simulink model "DCHR_Earliest_Dispatch_Stateflow_v79"  (R2026a)
settings: Solver=FixedStepDiscrete  StopTime=0  FixedStep=1
model workspace (MAT data in the model file):
  dispatch_cfg_v66 = [0 0.2 20 70 48 60 0.01 0.9 0.8 40 4 30 35 5 5 0.5 0.5 2 5 45 2 0.1 0.25 0.25 2 68]
  dispatch_input_v66 = [0 1 0 0.1 0 0.1 0 0 0 0 3 0 1]
settings Model: Creator=Lysda  LastModifiedBy=Lysda

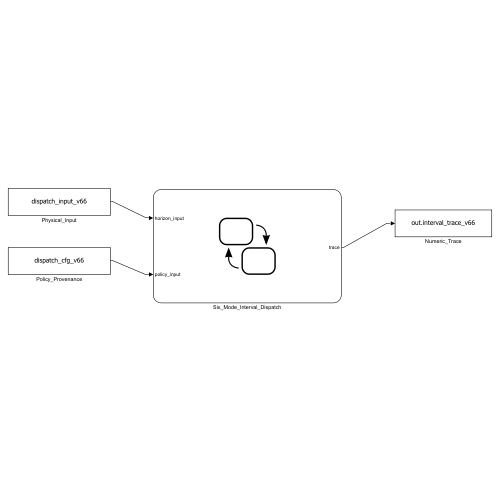
[thumbnail: Simulink's stored preview of the top-level diagram]
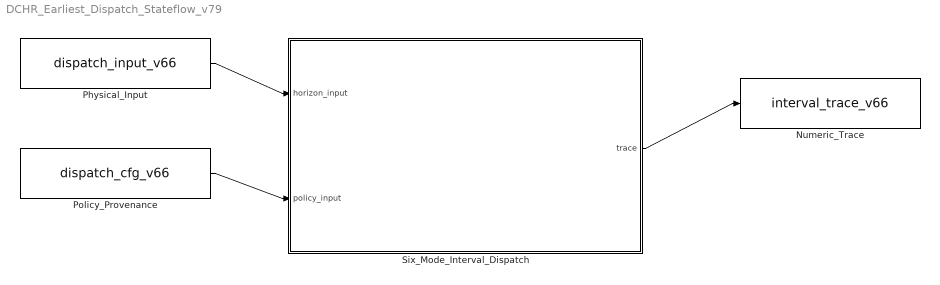
== system DCHR_Earliest_Dispatch_Stateflow_v79 ==
  Numeric_Trace : ToWorkspace  VariableName=interval_trace_v66  SaveFormat=Timeseries  SampleTime=-1
  Physical_Input : FromWorkspace  VariableName=dispatch_input_v66  SampleTime=1  Interpolate=off  OutputAfterFinalValue=Holding final value
  Policy_Provenance : FromWorkspace  VariableName=dispatch_cfg_v66  SampleTime=1  Interpolate=off  OutputAfterFinalValue=Holding final value
  Six_Mode_Interval_Dispatch : Stateflow chart  TreatAsAtomicUnit=on
  wires:
  Physical_Input/1 -> Six_Mode_Interval_Dispatch/1(horizon_input)
  Policy_Provenance/1 -> Six_Mode_Interval_Dispatch/2(policy_input)
  Six_Mode_Interval_Dispatch/1(trace) -> Numeric_Trace/1

== stateflow chart DCHR_Earliest_Dispatch_Stateflow_v79/Six_Mode_Interval_Dispatch ==
  settings: description=v79 pre-commit HP partition/energy/temporal-monitored SAME six-mode chart executes analytic earliest-event segments. Root hulls, symbolic thresholds, port offsets and physical clock survive each segment. No root midpoint. Macro solver ticks are protocol calls, not physical event times.
  state IDLE
    en:
    core=earliest_dispatch_kernel_v75(horizon_input,policy_input,retained_memory);
    assert(core(1)==0);
    monitor_hp_partition_v79(horizon_input,policy_input,retained_memory,core);
    trace=core;
    retained_memory=core;
    du:
    core=earliest_dispatch_kernel_v75(horizon_input,policy_input,retained_memory);
    assert(core(1)==0);
    monitor_hp_partition_v79(horizon_input,policy_input,retained_memory,core);
    trace=core;
    retained_memory=core;
  state HEAT_RECOVERY
    en:
    core=earliest_dispatch_kernel_v75(horizon_input,policy_input,retained_memory);
    assert(core(1)==1);
    monitor_hp_partition_v79(horizon_input,policy_input,retained_memory,core);
    trace=core;
    retained_memory=core;
    du:
    core=earliest_dispatch_kernel_v75(horizon_input,policy_input,retained_memory);
    assert(core(1)==1);
    monitor_hp_partition_v79(horizon_input,policy_input,retained_memory,core);
    trace=core;
    retained_memory=core;
  state STORAGE_CHARGE
    en:
    core=earliest_dispatch_kernel_v75(horizon_input,policy_input,retained_memory);
    assert(core(1)==2);
    monitor_hp_partition_v79(horizon_input,policy_input,retained_memory,core);
    trace=core;
    retained_memory=core;
    du:
    core=earliest_dispatch_kernel_v75(horizon_input,policy_input,retained_memory);
    assert(core(1)==2);
    monitor_hp_partition_v79(horizon_input,policy_input,retained_memory,core);
    trace=core;
    retained_memory=core;
  state STORAGE_DISCHARGE
    en:
    core=earliest_dispatch_kernel_v75(horizon_input,policy_input,retained_memory);
    assert(core(1)==3);
    monitor_hp_partition_v79(horizon_input,policy_input,retained_memory,core);
    trace=core;
    retained_memory=core;
    du:
    core=earliest_dispatch_kernel_v75(horizon_input,policy_input,retained_memory);
    assert(core(1)==3);
    monitor_hp_partition_v79(horizon_input,policy_input,retained_memory,core);
    trace=core;
    retained_memory=core;
  state BACKUP
    en:
    core=earliest_dispatch_kernel_v75(horizon_input,policy_input,retained_memory);
    assert(core(1)==4);
    monitor_hp_partition_v79(horizon_input,policy_input,retained_memory,core);
    trace=core;
    retained_memory=core;
    du:
    core=earliest_dispatch_kernel_v75(horizon_input,policy_input,retained_memory);
    assert(core(1)==4);
    monitor_hp_partition_v79(horizon_input,policy_input,retained_memory,core);
    trace=core;
    retained_memory=core;
  state UNMET_DEMAND
    en:
    core=earliest_dispatch_kernel_v75(horizon_input,policy_input,retained_memory);
    assert(core(1)==5);
    monitor_hp_partition_v79(horizon_input,policy_input,retained_memory,core);
    trace=core;
    retained_memory=core;
    du:
    core=earliest_dispatch_kernel_v75(horizon_input,policy_input,retained_memory);
    assert(core(1)==5);
    monitor_hp_partition_v79(horizon_input,policy_input,retained_memory,core);
    trace=core;
    retained_memory=core;
  (junction 60) -> UNMET_DEMAND [order 6] : [earliest_mode_v73(horizon_input,policy_input,retained_memory)==5]
  (junction 60) -> BACKUP [order 5] : [earliest_mode_v73(horizon_input,policy_input,retained_memory)==4]
  (junction 60) -> STORAGE_DISCHARGE [order 4] : [earliest_mode_v73(horizon_input,policy_input,retained_memory)==3]
  (junction 60) -> STORAGE_CHARGE [order 3] : [earliest_mode_v73(horizon_input,policy_input,retained_memory)==2]
  (junction 60) -> HEAT_RECOVERY [order 2] : [earliest_mode_v73(horizon_input,policy_input,retained_memory)==1]
  (default) -> (junction 60)
  (junction 60) -> IDLE [order 1] : [earliest_mode_v73(horizon_input,policy_input,retained_memory)==0]
  UNMET_DEMAND -> IDLE [order 1] : [earliest_mode_v73(horizon_input,policy_input,retained_memory)==0]
  BACKUP -> IDLE [order 1] : [earliest_mode_v73(horizon_input,policy_input,retained_memory)==0]
  STORAGE_DISCHARGE -> IDLE [order 1] : [earliest_mode_v73(horizon_input,policy_input,retained_memory)==0]
  STORAGE_CHARGE -> IDLE [order 1] : [earliest_mode_v73(horizon_input,policy_input,retained_memory)==0]
  HEAT_RECOVERY -> IDLE [order 1] : [earliest_mode_v73(horizon_input,policy_input,retained_memory)==0]
  UNMET_DEMAND -> HEAT_RECOVERY [order 2] : [earliest_mode_v73(horizon_input,policy_input,retained_memory)==1]
  BACKUP -> HEAT_RECOVERY [order 2] : [earliest_mode_v73(horizon_input,policy_input,retained_memory)==1]
  STORAGE_DISCHARGE -> HEAT_RECOVERY [order 2] : [earliest_mode_v73(horizon_input,policy_input,retained_memory)==1]
  STORAGE_CHARGE -> HEAT_RECOVERY [order 2] : [earliest_mode_v73(horizon_input,policy_input,retained_memory)==1]
  IDLE -> HEAT_RECOVERY [order 1] : [earliest_mode_v73(horizon_input,policy_input,retained_memory)==1]
  IDLE -> STORAGE_CHARGE [order 2] : [earliest_mode_v73(horizon_input,policy_input,retained_memory)==2]
  IDLE -> STORAGE_DISCHARGE [order 3] : [earliest_mode_v73(horizon_input,policy_input,retained_memory)==3]
  IDLE -> BACKUP [order 4] : [earliest_mode_v73(horizon_input,policy_input,retained_memory)==4]
  IDLE -> UNMET_DEMAND [order 5] : [earliest_mode_v73(horizon_input,policy_input,retained_memory)==5]
  UNMET_DEMAND -> STORAGE_CHARGE [order 3] : [earliest_mode_v73(horizon_input,policy_input,retained_memory)==2]
  BACKUP -> STORAGE_CHARGE [order 3] : [earliest_mode_v73(horizon_input,policy_input,retained_memory)==2]
  STORAGE_DISCHARGE -> STORAGE_CHARGE [order 3] : [earliest_mode_v73(horizon_input,policy_input,retained_memory)==2]
  HEAT_RECOVERY -> STORAGE_CHARGE [order 2] : [earliest_mode_v73(horizon_input,policy_input,retained_memory)==2]
  HEAT_RECOVERY -> STORAGE_DISCHARGE [order 3] : [earliest_mode_v73(horizon_input,policy_input,retained_memory)==3]
  HEAT_RECOVERY -> BACKUP [order 4] : [earliest_mode_v73(horizon_input,policy_input,retained_memory)==4]
  HEAT_RECOVERY -> UNMET_DEMAND [order 5] : [earliest_mode_v73(horizon_input,policy_input,retained_memory)==5]
  UNMET_DEMAND -> STORAGE_DISCHARGE [order 4] : [earliest_mode_v73(horizon_input,policy_input,retained_memory)==3]
  BACKUP -> STORAGE_DISCHARGE [order 4] : [earliest_mode_v73(horizon_input,policy_input,retained_memory)==3]
  STORAGE_CHARGE -> STORAGE_DISCHARGE [order 3] : [earliest_mode_v73(horizon_input,policy_input,retained_memory)==3]
  STORAGE_CHARGE -> BACKUP [order 4] : [earliest_mode_v73(horizon_input,policy_input,retained_memory)==4]
  STORAGE_CHARGE -> UNMET_DEMAND [order 5] : [earliest_mode_v73(horizon_input,policy_input,retained_memory)==5]
  UNMET_DEMAND -> BACKUP [order 5] : [earliest_mode_v73(horizon_input,policy_input,retained_memory)==4]
  STORAGE_DISCHARGE -> BACKUP [order 4] : [earliest_mode_v73(horizon_input,policy_input,retained_memory)==4]
  STORAGE_DISCHARGE -> UNMET_DEMAND [order 5] : [earliest_mode_v73(horizon_input,policy_input,retained_memory)==5]
  BACKUP -> UNMET_DEMAND [order 5] : [earliest_mode_v73(horizon_input,policy_input,retained_memory)==5]
  data: u function_input; p function_input; old function_input; y function_output; u function_input; cfg function_input; memory function_input; mode function_output; E function_input; B function_input; lambda function_input; target function_input; direction function_input; horizon function_input; dwell function_input; age function_input; z function_output; u function_input; p function_input; old function_input; y function_input; initial function_input; t function_input; lambda function_input; B function_input; en function_output; integral function_output; p function_input; horizon function_input; dwell function_input; age function_input; z function_output; u function_input; p function_input; old function_input; y function_input; u function_input; p function_input; old function_input; y function_input; horizon_input input double size=[12 1]; policy_input input double size=[25 1]; trace output double size=[1380 1]; retained_memory local double size=[1380 1] =zeros(1380,1); core local double size=[1380 1] =zeros(1380,1)
  function y=earliest_dispatch_kernel_v75(u,p,old):
    | function y=earliest_dispatch_kernel_v75(u,p,old)
    | %#codegen
    | % Interval-valued event segments with symbolic threshold contacts, never a
    | % root midpoint. See audit/Earliest_dispatch_derivation_v73.md for schema.
    | assert(all(isfinite([u;p;old])),'v73 finite domain');
    | assert(u(1)==1&&u(5)>0&&u(6)>=0&&u(7)>=0&&all(u(8:9)==0|u(8:9)==1),'v73 input domain');
    | assert(all(p([1 7 8 13 14 16 17 18])>0)&&p(7)<=1&&p(8)<=1&&p(6)>=0&& ...
    |     all(p([9 10 11 21 22 23 24])>=0)&&p(15)>0&&p(15)<=1,'v73 equipment domain');
    | assert(p(2)>-273.15&&p(2)<p(4)&&p(4)<p(5)&&p(5)<p(25)&&p(25)<p(3)&& ...
    |     p(19)<=p(4)&&p(6)*u(5)<=1,'v73 thermal/span domain');
    | P=@(v)[v v];C=P(p(1));Ta=P(p(2));cap=muliv(C,minusiv(P(p(3)),Ta));
    | cut=muliv(C,minusiv(P(p(4)),Ta));restart=muliv(C,minusiv(P(p(5)),Ta));stop=muliv(C,minusiv(P(p(25)),Ta));
    | y=zeros(1380,1);y(2)=75;y(73:75)=[u(5);u(7);u(8)+2*u(9)];y(76:100)=p;
    | if old(2)==0
    |     assert(u(10)>=0&&u(10)<cap(1)&&ismember(u(11),[0 1])&&u(12)>=0,'v73 initial domain');
    |     E=P(u(10));on=u(11);age=P(u(12));clock=P(0);tag=0;total=zeros(20,1);origin=E;ageCert=1;ageHi=u(12);ageErr=P(0);
    | else
    |     assert(old(2)==75&&all(old(76:100)==p),'v73 immutable policy');
    |     E=old(5:6)';on=old(7);age=old(8:9)';clock=old(10:11)';tag=old(12);total=old(31:50);origin=old(51:52)';ageCert=old(62);ageHi=old(63);ageErr=old(64:65)';
    | end
    | assert(E(1)>=0&&E(1)<=E(2)&&E(2)<cap(2)&&age(1)>=0&&age(1)<=age(2),'v73 retained bounds');
    | boundary=plusiv(clock,P(u(5)));assert(u(3)>clock(2)&&boundary(1)<=u(3)&&boundary(2)>=u(3),'v73 physical clock');
    | y(3:4)=E';y(51:52)=origin';y(58:59)=clock';y(60:61)=boundary';
    | Te=minusiv(minusiv(P(p(12)),P(p(13))),P(p(14)));a=muliv(P(p(15)),plusiv(Te,P(273.15)));
    | floor=plusiv(P(p(19)),P(p(20)));lf=minusiv(plusiv(floor,P(p(18))),Te);
    | assert(a(1)>0&&lf(1)>0,'v73 refrigerant domain');
    | sourceCap=muliv(P(u(7)),P(p(13)));
    | sourceLimit=muliv(sourceCap,plusiv(P(1),diviv(lf,a)));
    | waterLimit=muliv(P(p(16)),P(p(17)));
    | candidate=max(0,min([p(11),sourceLimit(1),waterLimit(1)]));
    | % Conservative binary allocation leaves room for the certified exact sum of
    | % separately rounded direct/charge ports. This is a power selection, not a
    | % relaxed physical guard or tolerance.
    | limit=max(0,candidate-8*eps(candidate));
    | y(66:71)=[sourceCap';sourceLimit';waterLimit'];
    | t=P(0);ports=zeros(20,1);finished=false;events=0;lastmode=0;
    | for slot=1:16
    |     assert(~finished,'v73 internal finished sequence');
    |     remaining=minusiv(P(u(5)),t);assert(remaining(1)>0,'v73 unresolved remaining duration');
    |     incoming=E;incomingAge=age;incomingOn=on;incomingTag=tag;
    |     potential=max(0,min(p(9),limit-min(u(6),limit)));
    |     belowStop=(tag==2||tag==3)||(tag==0&&E(2)<stop(1));
    |     canCharge=u(9)==1&&belowStop&&potential>0;
    |     request=u(6);if canCharge,request=request+potential;end
    |     sink=request>0;futureSink=u(6)>0||(u(9)==1&&potential>0);
    |     atRestart=tag==3||(tag==2)||(tag==0&&E(2)<=restart(1));
    |     reason=0;
    |     if on==1&&(limit==0||~sink),on=0;age=P(0);reason=3;
    |     elseif on==1&&u(8)==0
    |         assert(age(1)>=p(22)||(ageCert==1&&certifiedAge(ageHi,ageErr,p(22))),'v73 ON dwell not certified');on=0;age=P(0);reason=2;
    |     elseif on==0&&u(8)==1&&limit>0&&sink&&atRestart&&age(1)>=p(23)
    |         on=1;age=P(0);reason=1;
    |     end
    |     hp=0;if on==1,hp=min(request,limit);end
    |     direct=min(u(6),hp);charge=0;if canCharge,charge=min(potential,max(0,hp-direct));end
    |     dis=0;aboveCut=tag==1||tag==3||(tag==0&&E(1)>cut(2));
    |     if charge==0&&aboveCut,dis=min(p(10),max(0,u(6)-direct));end
    |     boiler=min(p(24),max(0,u(6)-direct-dis));unmet=max(0,u(6)-direct-dis-boiler);
    |     B=minusiv(muliv(P(p(7)),P(charge)),diviv(P(dis),P(p(8))));
    |     mode=0;if unmet>0,mode=5;elseif boiler>0,mode=4;elseif dis>0,mode=3;elseif charge>0,mode=2;elseif direct>0,mode=1;end
    |     candidates=zeros(3,15);enabled=[charge>0 dis>0 on==0&&u(8)==1&&limit>0&&futureSink];
    |     if enabled(1)
    |         deriv=minusiv(B,muliv(P(p(6)),stop));
    |         if deriv(1)>0,candidates(1,:)=certify_event_root_v73(E,B,p(6),stop,1,u(5),0,P(0))';
    |         elseif deriv(2)>0,assert(false,'v73 unresolved stop derivative');end
    |     end
    |     if enabled(2),candidates(2,:)=certify_event_root_v73(E,B,p(6),cut,-1,u(5),0,P(0))';end
    |     if enabled(3)
    |         if atRestart
    |             r=zeros(1,15);r(1)=3;r(8:9)=max(0,minusiv(P(p(23)),age));r(10:11)=r(8:9);r(13)=-1;r(14:15)=restart;candidates(3,:)=r;
    |         else
    |             deriv=minusiv(B,muliv(P(p(6)),restart));
    |             if tag==1&&all(B==0)&&p(6)>0&&p(25)-p(5)<=.5*(p(5)-p(2))
    |                 candidates(3,:)=passive_contact_root_v73r2(p,u(5),p(23),age)';y(72)=1;
    |             elseif deriv(2)<0,candidates(3,:)=certify_event_root_v73(E,B,p(6),restart,-1,u(5),p(23),age)';
    |             elseif deriv(1)<0,assert(false,'v73 unresolved restart derivative');end
    |         end
    |     end
    |     duration=remaining;event=0;
    |     for j=1:3
    |         r=candidates(j,:);if r(1)==0,continue;end
    |         if r(1)==2
    |             % An unresolved root at the original macro span is harmless only
    |             % if the entire actual remaining trajectory is certainly before it.
    |             [tail,~]=flow(E,remaining,p(6),B);
    |             if j==1,before=tail(2)<stop(1);elseif j==2,before=tail(1)>cut(2);else,before=tail(1)>restart(2);end
    |             assert(before,'v73 unresolved event boundary');continue;
    |         end
    |         ready=r(10:11);
    |         if ready(1)>remaining(2),continue;end
    |         assert(ready(2)<remaining(1),'v73 unresolved event boundary');
    |         if event==0||ready(2)<duration(1),duration=ready;event=j;
    |         elseif ready(1)<=duration(2),assert(false,'v73 unresolved enabled event ordering');end
    |     end
    |     assert(duration(1)>0,'v73 zero-progress event');
    |     [endpoint,integral]=flow(E,duration,p(6),B);newtag=0;thermal=0;
    |     if event==1,endpoint=stop;newtag=1;thermal=1;
    |     elseif event==2,endpoint=cut;newtag=2;thermal=1;
    |     elseif event==3
    |         r=candidates(3,:);
    |         if r(1)==1&&r(2)>r(9),endpoint=restart;newtag=3;thermal=1;
    |         elseif r(8)>r(3)||r(1)==3
    |             % The age identity age+(minOFF-age)=minOFF is retained,
    |             % not reconstructed from independent interval endpoints.
    |             assert(endpoint(2)<=restart(2)||atRestart,'v73 dwell thermal readiness');
    |         else,assert(false,'v73 unresolved thermal/dwell ordering');end
    |         if thermal==1,assert(plusiv(age,duration)*[1;0]>=p(23),'v73 OFF dwell not certified');end
    |     end
    |     assert(endpoint(1)>=0&&endpoint(2)<cap(2),'v73 TES bounds');
    |     assert(dis==0||event==2||endpoint(1)>=cut(2),'v73 discharge cutoff');
    |     assert(charge==0||event==1||endpoint(2)<stop(1),'v73 charging stop');
    |     % The source rectangles cover the full event duration box. The exact
    |     % root/threshold relation is recorded; Cartesian evaluation only widens it.
    |     q=plusiv(P(direct),P(charge));src=P(0);work=P(0);
    |     % q <= S*(1+liftFloor/a), hot >= floor, a>0 imply source<=S.
    |     % Retain this relation instead of demanding disjoint widened boxes.
    |     assert(q(2)<=sourceLimit(1)&&q(2)<=waterLimit(1)&&q(2)<=p(11),'v73 selected power certificate');
    |     for cell=1:32
    |         t0=muliv(duration,P((cell-1)/32));t1=muliv(duration,P(cell/32));
    |         [e0,~]=flow(E,t0,p(6),B);[e1,~]=flow(E,t1,p(6),B);
    |         eh=[min(e0(1),e1(1)) max(e0(2),e1(2))];hot=plusiv(plusiv(Ta,diviv(eh,C)),P(p(17)));
    |         hot=[max(floor(1),hot(1)) max(floor(2),hot(2))];lift=minusiv(plusiv(hot,P(p(18))),Te);
    |         rate=muliv(q,diviv(a,plusiv(a,lift)));
    |         assert(lift(1)>0,'v73 positive work lift');
    |         % Intersection is justified by the selected-power/floor certificate.
    |         rate=[max(0,rate(1)) min(sourceCap(2),rate(2))];
    |         assert(rate(1)<=rate(2),'v73 finite source certificate intersection');
    |         wrate=muliv(q,diviv(lift,plusiv(a,lift)));
    |         work=plusiv(work,muliv(wrate,diviv(duration,P(32))));
    |         src=plusiv(src,muliv(rate,diviv(duration,P(32))));
    |     end
    |     assert(q(2)<=muliv(P(p(16)),P(p(17)))*[0;1],'v73 finite water capacity');
    |     heat=muliv(q,duration);standing=muliv(P(p(6)),integral);
    |     closs=muliv(minusiv(P(1),P(p(7))),muliv(P(charge),duration));
    |     dloss=muliv(minusiv(diviv(P(1),P(p(8))),P(1)),muliv(P(dis),duration));
    |     service=muliv(P(direct+dis+boiler),duration);back=muliv(P(boiler),duration);missing=muliv(P(unmet),duration);aux=muliv(P(p(21)),work);
    |     increment=[heat';src';work';standing';closs';dloss';service';back';missing';aux'];
    |     assert(all(increment>=0),'v73 nonnegative energy');
    |     seglaw=minusiv(minusiv(minusiv(minusiv(plusiv(E,plusiv(heat,back)),service),endpoint),standing),plusiv(closs,dloss));
    |     assert(seglaw(1)<=0&&seglaw(2)>=0,'v73 segment first law');
    |     offset=ports;for j=1:10,ix=2*j-1:2*j;ports(ix)=plusiv(ports(ix)',increment(ix)')';end
    |     elapsed=plusiv(t,duration);newage=plusiv(age,duration);outOn=on;
    |     if event==1,outOn=0;newage=P(0);elseif event==3,outOn=1;newage=P(0);end
    |     z=zeros(80,1);z(1:4)=[slot;mode;event;thermal];z(5:6)=t';z(7:8)=duration';z(9:10)=elapsed';
    |     z(11:14)=[E';endpoint'];z(15:18)=[age';newage'];z(19:23)=[on;outOn;incomingTag;newtag;reason];
    |     z(24:29)=[hp;direct;charge;dis;boiler;unmet];z(30:31)=B';z(32:51)=increment;z(52:71)=offset;
    |     if event>0,z(72:73)=candidates(event,2:3)';z(74:75)=candidates(event,8:9)';z(76:77)=candidates(event,14:15)';end
    |     z(78:80)=[incomingOn;incomingAge'];y(100+80*(slot-1)+(1:80))=z;
    |     % Exact binary macro durations admit a compensated age identity only
    |     % when no uncertain event intervened. Event ages keep their hull alone.
    |     if slot==1&&event==0
    |         if reason~=0,ageCert=1;ageHi=0;ageErr=P(0);end
    |         if ageCert==1,[ageHi,e]=twoSum(ageHi,u(5));ageErr=plusiv(ageErr,P(e));end
    |     else,ageCert=0;ageHi=0;ageErr=P(0);end
    |     E=endpoint;on=outOn;age=newage;tag=newtag;lastmode=mode;t=elapsed;
    |     if event==0
    |         % Exact held boundary identity t_start+(dt-t_start)=dt, with its
    |         % expression recorded in duration/offset fields. No midpoint used.
    |         t=P(u(5));finished=true;y(13)=slot;break;
    |     else,events=events+1;end
    | end
    | assert(finished,'v73 event segment budget');
    | for j=1:10,ix=2*j-1:2*j;total(ix)=plusiv(total(ix)',ports(ix)')';end
    | law=minusiv(minusiv(minusiv(minusiv(plusiv(origin,plusiv(total(1:2)',total(15:16)')),total(13:14)'),E),total(7:8)'),plusiv(total(9:10)',total(11:12)'));
    | assert(law(1)<=0&&law(2)>=0,'v73 cumulative first law');
    | y(1)=lastmode;y(5:6)=E';y(7)=on;y(8:9)=age';y(10:11)=boundary';y(12)=tag;y(14)=events;
    | y(15:30)=ports(1:16);y(31:50)=total;y(53:54)=law';y(55:56)=ports(17:18);y(57)=limit;y(62:65)=[ageCert;ageHi;ageErr'];
    | end
    | function [en,integral]=flow(initial,t,lambda,B)
    | [en,integral]=inventory_flow_v73(initial,t,lambda,B);
    | end
    | function ok=certifiedAge(hi,err,minimum)
    | [s,e]=twoSum(hi,-minimum);delta=plusiv([s s],plusiv([e e],err));ok=delta(1)>=0;
    | end
    | function [s,e]=twoSum(a,b)
    | s=a+b;bb=s-a;e=(a-(s-bb))+(b-bb);
    | assert(isfinite(s)&&isfinite(e),'v73 age certificate overflow');
    | end
    | function z=plusiv(x,y)
    | if all(x==0),z=y;elseif all(y==0),z=x;
    | elseif x(1)==x(2)&&y(1)==y(2)&&x(1)==-y(1),z=[0 0];
    | else,z=out([x(1)+y(1) x(2)+y(2)]);end
    | end
    | function z=minusiv(x,y)
    | if all(y==0),z=x;elseif x(1)==x(2)&&y(1)==y(2)&&x(1)==y(1),z=[0 0];else,z=out([x(1)-y(2) x(2)-y(1)]);end
    | end
    | function z=muliv(x,y)
    | if all(x==0)||all(y==0),z=[0 0];return;end
    | t=[x(1)*y(1) x(1)*y(2) x(2)*y(1) x(2)*y(2)];z=out([min(t) max(t)]);
    | end
    | function z=diviv(x,y)
    | assert(y(1)>0,'v73 positive denominator');if all(x==0),z=[0 0];return;end
    | if x(1)==x(2)&&y(1)==y(2)&&x(1)==y(1),z=[1 1];return;end
    | t=[x(1)/y(1) x(1)/y(2) x(2)/y(1) x(2)/y(2)];z=out([min(t) max(t)]);
    | end
    | function z=out(t)
    | assert(all(isfinite(t)),'v73 arithmetic overflow');z=[t(1)-2*eps(t(1)) t(2)+2*eps(t(2))];assert(all(isfinite(z)),'v73 outward overflow');
    | end
  function mode=earliest_mode_v73(u,cfg,memory):
    | function mode=earliest_mode_v73(u,cfg,memory)
    | y=earliest_dispatch_kernel_v75(u,cfg,memory);mode=y(1);
    | end
  function z=certify_event_root_v73(E,B,lambda,target,direction,horizon,dwell,age):
    | function z=certify_event_root_v73(E,B,lambda,target,direction,horizon,dwell,age)
    | %#codegen
    | % Held affine trajectory certificate. This returns a bracket, never a state reset.
    | % z=[status,tlo,thi,E(tlo).lo,hi,E(thi).lo,hi,wait.lo,hi,
    | %    ready.lo,hi,ordering,direction,target.lo,hi].
    | % status: 0 no crossing in horizon, 1 strict interior bracket,
    | % 2 unresolved contact/horizon, 3 already on the reached side.
    | % ordering: 0 no event, 1 ready strictly before horizon,
    | % 2 ordering unresolved, 3 ready strictly after horizon.
    | assert(all(isfinite([E B lambda target direction horizon dwell age])), 'v67 finite root domain');
    | assert(E(1)>=0&&E(1)<=E(2)&&B(1)<=B(2)&&target(1)>=0&&target(1)<=target(2)&& ...
    |     lambda>=0&&horizon>0&&lambda*horizon<=1&&ismember(direction,[-1 1])&& ...
    |     dwell>=0&&age(1)>=0&&age(1)<=age(2),'v67 root domain');
    | P=@(x)[x x];z=zeros(15,1);z(13)=direction;z(14:15)=target';
    | wait=minusiv(P(dwell),age);wait=max(0,wait);z(8:9)=wait';
    | before=@(v) (direction==1&&v(2)<target(1))||(direction==-1&&v(1)>target(2));
    | after=@(v) (direction==1&&v(1)>target(2))||(direction==-1&&v(2)<target(1));
    | reached=(direction==1&&E(1)>=target(2))||(direction==-1&&E(2)<=target(1));
    | if reached
    |     z(1)=3;z(4:7)=[E';E'];z(10:11)=wait';
    | elseif ~before(E)
    |     z(1)=2;z(2:3)=[0;horizon];z(12)=2;return;
    | else
    |     % Derivative sign at both ends certifies monotonicity on the entire
    |     % reachable segment. Equilibria and unresolved monotonicity are refused.
    |     d0=minusiv(B,muliv(P(lambda),E));d1=minusiv(B,muliv(P(lambda),target));
    |     if direction==1
    |         assert(d0(1)>0&&d1(1)>0,'v67 increasing root not certified');
    |     else
    |         assert(d0(2)<0&&d1(2)<0,'v67 decreasing root not certified');
    |     end
    |     endpoint=flow(E,P(horizon),lambda,B);
    |     if before(endpoint)
    |         z(1)=0;z(2:3)=horizon;z(4:7)=[endpoint';endpoint'];return;
    |     elseif ~after(endpoint)
    |         z(1)=2;z(2:3)=[0;horizon];z(4:7)=[E';endpoint'];z(12)=2;return;
    |     end
    |     % Search for the latest certainly-before and earliest certainly-after
    |     % witnesses independently. Ambiguous evaluations never choose a side.
    |     lo=0;right=horizon;
    |     for j=1:48
    |         mid=lo+(right-lo)/2;v=flow(E,P(mid),lambda,B);
    |         if before(v),lo=mid;else,right=mid;end
    |     end
    |     left=0;hi=horizon;
    |     for j=1:48
    |         mid=left+(hi-left)/2;v=flow(E,P(mid),lambda,B);
    |         if after(v),hi=mid;else,left=mid;end
    |     end
    |     elo=flow(E,P(lo),lambda,B);ehi=flow(E,P(hi),lambda,B);
    |     assert(before(elo)&&after(ehi)&&0<=lo&&lo<hi&&hi<horizon,'v67 root witnesses');
    |     z(1)=1;z(2:3)=[lo;hi];z(4:7)=[elo';ehi'];
    |     z(10:11)=[max(lo,wait(1));max(hi,wait(2))];
    | end
    | if z(11)<horizon,z(12)=1;elseif z(10)>horizon,z(12)=3;else,z(12)=2;end
    | end
    | function en=flow(initial,t,lambda,B)
    | [en,~]=inventory_flow_v73(initial,t,lambda,B);
    | end
    | function z=plusiv(x,y)
    | if all(x==0),z=y;elseif all(y==0),z=x;else,z=out([x(1)+y(1) x(2)+y(2)]);end
    | end
    | function z=minusiv(x,y)
    | if all(y==0),z=x;elseif x(1)==x(2)&&y(1)==y(2)&&x(1)==y(1),z=[0 0];else,z=out([x(1)-y(2) x(2)-y(1)]);end
    | end
    | function z=muliv(x,y)
    | if all(x==0)||all(y==0),z=[0 0];return;end
    | t=[x(1)*y(1) x(1)*y(2) x(2)*y(1) x(2)*y(2)];z=out([min(t) max(t)]);
    | end
    | function z=diviv(x,y)
    | assert(y(1)>0,'v67 positive root denominator');
    | if all(x==0),z=[0 0];return;end
    | t=[x(1)/y(1) x(1)/y(2) x(2)/y(1) x(2)/y(2)];z=out([min(t) max(t)]);
    | end
    | function z=out(t)
    | assert(all(isfinite(t)),'v67 root arithmetic overflow');z=[t(1)-2*eps(t(1)) t(2)+2*eps(t(2))];
    | assert(all(isfinite(z))&&z(1)<=z(2),'v67 root expansion overflow');
    | end
  function monitor_temporal_commit_v77(u,p,old,y):
    | function monitor_temporal_commit_v77(u,p,old,y)
    | %#codegen
    | % Verify the candidate record BEFORE trace emission and retained-memory commit.
    | % Trace schema remains 75; model release is 77. No thermal solver is called.
    | assert(all(isfinite(y))&&y(2)==75&&all(y(76:100)==p),'v77 schema');
    | assert(y(13)>=1&&y(13)<=16&&y(13)==fix(y(13)),'v77 segment count');
    | assert(all(y(100+80*y(13)+1:end)==0),'v77 unused segments');
    | assert(all(y(73:75)==[u(5);u(7);u(8)+2*u(9)]),'v77 input binding');
    | if old(2)==0
    |     E=[u(10) u(10)];on=u(11);age=[u(12) u(12)];tag=0;clock=[0 0];
    | else
    |     assert(old(2)==75&&all(old(76:100)==p),'v77 retained schema');
    |     E=old(5:6)';on=old(7);age=old(8:9)';tag=old(12);clock=old(10:11)';
    | end
    | boundary=plusiv(clock,[u(5) u(5)]);
    | assert(all(y(3:4)'==E)&&all(y(58:59)'==clock)&& ...
    |     all(y(60:61)'==boundary)&&all(y(10:11)'==boundary),'v77 macro continuity');
    | t=[0 0];events=0;mode=0;
    | for j=1:y(13)
    |     z=y(100+80*(j-1)+(1:80));d=z(7:8)';event=z(3);reason=z(23);
    |     assert(d(1)>0&&d(1)<=d(2)&&ismember(event,0:3)&& ...
    |         ismember(reason,0:3)&&ismember(z(4),[0 1]),'v77 transition domain');
    |     assert(all(z(5:6)'==t)&&all(z(9:10)'==plusiv(t,d)),'v77 segment clock');
    |     assert(all(z(11:12)'==E)&&z(78)==on&&all(z(79:80)'==age)&&z(21)==tag,'v77 incoming memory');
    |     currentOn=on;currentAge=age;
    |     if reason>0
    |         assert((reason==1&&on==0)||(reason>=2&&on==1),'v77 boundary transition');
    |         currentAge=[0 0];currentOn=double(reason==1);
    |     end
    |     assert(z(19)==currentOn&&all(z(15:16)'==currentAge),'v77 boundary memory');
    |     nextOn=currentOn;nextAge=plusiv(currentAge,d);nextTag=0;
    |     if event==1,nextOn=0;nextAge=[0 0];nextTag=1;
    |     elseif event==2,nextTag=2;
    |     elseif event==3,nextOn=1;nextAge=[0 0];nextTag=3*z(4);end
    |     assert(z(20)==nextOn&&all(z(17:18)'==nextAge)&&z(22)==nextTag&& ...
    |         ((event==0&&z(4)==0)||(event==1&&z(4)==1)||(event==2&&z(4)==1)||event==3),'v77 event memory');
    |     if j==y(13)
    |         assert(event==0&&all(d==minusiv([u(5) u(5)],t)),'v77 held boundary');
    |     else
    |         assert(event>0,'v77 interior event');
    |     end
    |     E=z(13:14)';on=nextOn;age=nextAge;tag=nextTag;t=z(9:10)';
    |     events=events+double(event>0);mode=z(2);
    | end
    | assert(all(y(5:6)'==E)&&y(7)==on&&all(y(8:9)'==age)&&y(12)==tag,'v77 endpoint memory');
    | assert(y(1)==mode&&y(14)==events,'v77 mode event count');
    | end
    | function z=plusiv(x,y)
    | if all(x==0),z=y;elseif all(y==0),z=x;
    | elseif x(1)==x(2)&&y(1)==y(2)&&x(1)==-y(1),z=[0 0];
    | else,z=out([x(1)+y(1) x(2)+y(2)]);end
    | end
    | function z=minusiv(x,y)
    | if all(y==0),z=x;elseif x(1)==x(2)&&y(1)==y(2)&&x(1)==y(1),z=[0 0];
    | else,z=out([x(1)-y(2) x(2)-y(1)]);end
    | end
    | function z=out(x)
    | z=[x(1)-2*eps(x(1)) x(2)+2*eps(x(2))];
    | assert(all(isfinite(z)),'v77 temporal arithmetic');
    | end
  function [en,integral]=inventory_flow_v73(initial,t,lambda,B):
    | function [en,integral]=inventory_flow_v73(initial,t,lambda,B)
    | %#codegen
    | % Monotone affine inventory image. Exact E and B dependence occurs once.
    | % Each corner is monotone in time (its derivative has constant sign).
    | % Positive Taylor exp(+lambda*t), followed by reciprocal, avoids passive
    | % subtraction/wrapping. All arithmetic bounds expand by two binary ulps.
    | assert(initial(1)>=0&&initial(1)<=initial(2)&&t(1)>=0&&t(1)<=t(2)&& ...
    |     lambda>=0&&lambda*t(2)<=2&&B(1)<=B(2),'v73 flow domain');
    | if all(t==0),en=initial;integral=[0 0];return;end
    | lo=zeros(1,4);hi=zeros(1,4);n=0;
    | for ei=1:2
    |     for ti=1:2
    |         n=n+1;[value,~]=corner(initial(ei),t(ti),lambda,B(ei));lo(n)=value(1);hi(n)=value(2);
    |     end
    | end
    | en=[min(lo) max(hi)];
    | % Integral's positive trajectory has monotone initial/forcing dependence;
    | % its direct phi image remains conservative for variable time.
    | [~,f1,f2]=coeff(t,lambda);
    | integral=plusiv(muliv(initial,muliv(t,f1)),muliv(B,muliv(muliv(t,t),f2)));
    | end
    | function [en,unused]=corner(E,t,lambda,B)
    | P=@(x)[x x];[r,f1,~]=coeff(P(t),lambda);
    | if t==0,en=P(E);
    | elseif B==0,en=muliv(P(E),r);
    | else
    |     % Singleton corner evaluation retains small active changes without
    |     % subtracting rounded exponential factors. Uncertain inventory is never
    |     % used twice as independent operands: its monotone corners are separate.
    |     v=plusiv(muliv(P(-lambda),P(E)),P(B));
    |     en=plusiv(P(E),muliv(muliv(v,P(t)),f1));
    | end
    | unused=0;
    | end
    | function [r,f1,f2]=coeff(t,lambda)
    | P=@(x)[x x];
    | if lambda==0,r=P(1);f1=P(1);f2=P(.5);return;end
    | x=muliv(P(lambda),t);term=P(1);ex=P(1);
    | for j=1:30,term=diviv(muliv(term,x),P(j));ex=plusiv(ex,term);end
    | fac=P(1);for j=2:31,fac=muliv(fac,P(j));end
    | % e^2<8; positive-series remainder <=8*2^31/31! on [0,2].
    | tail=diviv(P(17179869184),fac);ex=plusiv(ex,[0 tail(2)]);r=diviv(P(1),ex);
    | x=-[x(2) x(1)];term=P(1);f1=P(1);f2=P(.5);
    | for j=1:24,term=diviv(muliv(term,x),P(j+1));f1=plusiv(f1,term);f2=plusiv(f2,diviv(term,P(j+2)));end
    | fac=P(1);for j=2:26,fac=muliv(fac,P(j));end
    | tail=diviv(P(268435456),fac);f1=plusiv(f1,[-tail(2) tail(2)]);f2=plusiv(f2,[-tail(2) tail(2)]);
    | end
    | function z=plusiv(x,y)
    | if all(x==0),z=y;elseif all(y==0),z=x;else,z=out([x(1)+y(1) x(2)+y(2)]);end
    | end
    | function z=muliv(x,y)
    | if all(x==0)||all(y==0),z=[0 0];return;end
    | t=[x(1)*y(1) x(1)*y(2) x(2)*y(1) x(2)*y(2)];z=out([min(t) max(t)]);
    | end
    | function z=diviv(x,y)
    | assert(y(1)>0,'v73 flow denominator');if all(x==0),z=[0 0];return;end
    | t=[x(1)/y(1) x(1)/y(2) x(2)/y(1) x(2)/y(2)];z=out([min(t) max(t)]);
    | end
    | function z=out(t)
    | assert(all(isfinite(t)),'v73 flow overflow');z=[t(1)-2*eps(t(1)) t(2)+2*eps(t(2))];
    | assert(all(isfinite(z)),'v73 flow outward overflow');
    | end
  function z=passive_contact_root_v73r2(p,horizon,dwell,age):
    | function z=passive_contact_root_v73r2(p,horizon,dwell,age)
    | %#codegen
    | % Exact symbolic STOP -> RESTART contact, B=0. The common heat capacity
    | % cancels: tau=log1p((Tstop-Trestart)/(Trestart-Ta))/lambda.
    | % This applies only with the retained STOP tag, never to a general E box.
    | P=@(v)[v v];assert(p(6)>0&&p(25)>p(5)&&p(5)>p(2),'v73r2 passive contact domain');
    | difference=minusiv(P(p(25)),P(p(5)));base=minusiv(P(p(5)),P(p(2)));
    | x=diviv(difference,base);assert(x(1)>0&&x(2)<=.5,'v73r2 log1p domain');
    | term=x;value=x;
    | for j=2:32
    |     term=muliv(term,x);part=diviv(term,P(j));
    |     if mod(j,2)==0,value=minusiv(value,part);else,value=plusiv(value,part);end
    | end
    | % Alternating log series error <=x^33/33 for 0<x<=1/2.
    | tail=diviv(muliv(term,x),P(33));value=plusiv(value,[0 tail(2)]);
    | time=diviv(value,P(p(6)));wait=max(0,minusiv(P(dwell),age));ready=max(time,wait);
    | target=muliv(P(p(1)),minusiv(P(p(5)),P(p(2))));
    | z=zeros(15,1);z(13)=-1;z(14:15)=target';z(8:9)=wait';z(10:11)=ready';z(2:3)=time';
    | if time(1)>horizon
    |     z(1)=0;z(12)=3;
    | elseif time(2)>=horizon
    |     z(1)=2;z(12)=2;
    | else
    |     z(1)=1;
    |     if ready(2)<horizon,z(12)=1;elseif ready(1)>horizon,z(12)=3;else,z(12)=2;end
    | end
    | end
    | function z=plusiv(x,y)
    | if all(x==0),z=y;elseif all(y==0),z=x;else,z=out([x(1)+y(1) x(2)+y(2)]);end
    | end
    | function z=minusiv(x,y)
    | if all(y==0),z=x;else,z=out([x(1)-y(2) x(2)-y(1)]);end
    | end
    | function z=muliv(x,y)
    | if all(x==0)||all(y==0),z=[0 0];return;end
    | v=[x(1)*y(1) x(1)*y(2) x(2)*y(1) x(2)*y(2)];z=out([min(v) max(v)]);
    | end
    | function z=diviv(x,y)
    | assert(y(1)>0,'v73r2 positive contact denominator');if all(x==0),z=[0 0];return;end
    | v=[x(1)/y(1) x(1)/y(2) x(2)/y(1) x(2)/y(2)];z=out([min(v) max(v)]);
    | end
    | function z=out(v)
    | assert(all(isfinite(v)),'v73r2 contact overflow');z=[v(1)-2*eps(v(1)) v(2)+2*eps(v(2))];
    | end
  function monitor_energy_commit_v78(u,p,old,y):
    | function monitor_energy_commit_v78(u,p,old,y)
    | %#codegen
    | % Candidate energy/port verification before emission and retained-state commit.
    | % v77 checks schema/count/temporal links first. No thermal solver is called here.
    | monitor_temporal_commit_v77(u,p,old,y);
    | ports=zeros(20,1);total=zeros(20,1);origin=[u(10) u(10)];
    | if old(2)~=0,total=old(31:50);origin=old(51:52)';end
    | assert(all(y(51:52)'==origin),'v78 origin binding');
    | cap=muliv([p(1) p(1)],minusiv([p(3) p(3)],[p(2) p(2)]));
    | assert(y(57)>=0&&y(57)<=p(11)&&y(57)<=y(68)&&y(57)<=y(70),'v78 selected capacity');
    | for j=1:y(13)
    |     z=y(100+80*(j-1)+(1:80));d=z(7:8)';q=z(24:29);inc=z(32:51);
    |     assert(z(1)==j&&ismember(z(2),0:5)&&all(q>=0),'v78 port domain');
    |     assert(q(1)<=y(57)&&q(3)<=p(9)&&q(4)<=p(10)&&q(5)<=p(24)&& ...
    |         (q(3)==0||q(4)==0)&&(z(19)==1||q(1)==0),'v78 port capacity');
    |     heatPower=plusiv([q(2) q(2)],[q(3) q(3)]);
    |     assert(heatPower(1)<=q(1)&&q(1)<=heatPower(2),'v78 HP allocation');
    |     servicePower=plusiv(plusiv([q(2) q(2)],[q(4) q(4)]),[q(5) q(5)]);
    |     allocation=plusiv(servicePower,[q(6) q(6)]);
    |     assert(allocation(1)<=u(6)&&u(6)<=allocation(2),'v78 demand allocation');
    |     expectedMode=0;
    |     if q(6)>0,expectedMode=5;elseif q(5)>0,expectedMode=4;elseif q(4)>0,expectedMode=3;
    |     elseif q(3)>0,expectedMode=2;elseif q(2)>0,expectedMode=1;end
    |     assert(z(2)==expectedMode,'v78 mode allocation');
    |     assert(z(11)>=0&&z(11)<=z(12)&&z(12)<cap(2)&& ...
    |         z(13)>=0&&z(13)<=z(14)&&z(14)<cap(2),'v78 TES domain');
    |     B=minusiv(muliv([p(7) p(7)],[q(3) q(3)]),diviv([q(4) q(4)],[p(8) p(8)]));
    |     assert(all(z(30:31)'==B),'v78 forcing binding');
    |     assert(all(inc>=0)&&all(inc(1:2:end)<=inc(2:2:end)),'v78 energy domain');
    |     assert(all(z(52:71)==ports),'v78 segment offsets');
    |     heat=muliv(heatPower,d);service=muliv([q(2)+q(4)+q(5) q(2)+q(4)+q(5)],d);
    |     back=muliv([q(5) q(5)],d);missing=muliv([q(6) q(6)],d);
    |     assert(all(inc(1:2)'==heat)&&all(inc(13:14)'==service)&& ...
    |         all(inc(15:16)'==back)&&all(inc(17:18)'==missing),'v78 port energy binding');
    |     closs=muliv(minusiv([1 1],[p(7) p(7)]),muliv([q(3) q(3)],d));
    |     dloss=muliv(minusiv(diviv([1 1],[p(8) p(8)]),[1 1]),muliv([q(4) q(4)],d));
    |     assert(all(inc(9:10)'==closs)&&all(inc(11:12)'==dloss),'v78 efficiency loss binding');
    |     sourceWork=plusiv(inc(3:4)',inc(5:6)');
    |     assert(sourceWork(1)<=heat(2)&&heat(1)<=sourceWork(2),'v78 HP first law');
    |     assert(all(inc(19:20)'==muliv([p(21) p(21)],inc(5:6)')),'v78 auxiliary binding');
    |     law=minusiv(minusiv(minusiv(minusiv(plusiv(z(11:12)',plusiv(heat,back)),service),z(13:14)'),inc(7:8)'),plusiv(closs,dloss));
    |     assert(law(1)<=0&&law(2)>=0,'v78 segment first law');
    |     for k=1:10,ix=2*k-1:2*k;ports(ix)=plusiv(ports(ix)',inc(ix)')';end
    | end
    | assert(all(y(15:30)==ports(1:16))&&all(y(55:56)==ports(17:18)),'v78 interval totals');
    | for k=1:10,ix=2*k-1:2*k;total(ix)=plusiv(total(ix)',ports(ix)')';end
    | assert(all(y(31:50)==total),'v78 cumulative totals');
    | law=minusiv(minusiv(minusiv(minusiv(plusiv(origin,plusiv(total(1:2)',total(15:16)')),total(13:14)'),y(5:6)'),total(7:8)'),plusiv(total(9:10)',total(11:12)'));
    | assert(all(y(53:54)'==law)&&law(1)<=0&&law(2)>=0,'v78 cumulative first law');
    | end
    | function z=plusiv(x,y)
    | if all(x==0),z=y;elseif all(y==0),z=x;
    | elseif x(1)==x(2)&&y(1)==y(2)&&x(1)==-y(1),z=[0 0];
    | else,z=out([x(1)+y(1) x(2)+y(2)]);end
    | end
    | function z=minusiv(x,y)
    | if all(y==0),z=x;elseif x(1)==x(2)&&y(1)==y(2)&&x(1)==y(1),z=[0 0];
    | else,z=out([x(1)-y(2) x(2)-y(1)]);end
    | end
    | function z=muliv(x,y)
    | if all(x==0)||all(y==0),z=[0 0];return;end
    | t=[x(1)*y(1) x(1)*y(2) x(2)*y(1) x(2)*y(2)];z=out([min(t) max(t)]);
    | end
    | function z=diviv(x,y)
    | assert(y(1)>0,'v78 positive denominator');if all(x==0),z=[0 0];return;end
    | if x(1)==x(2)&&y(1)==y(2)&&x(1)==y(1),z=[1 1];return;end
    | t=[x(1)/y(1) x(1)/y(2) x(2)/y(1) x(2)/y(2)];z=out([min(t) max(t)]);
    | end
    | function z=out(x)
    | z=[x(1)-2*eps(x(1)) x(2)+2*eps(x(2))];assert(all(isfinite(z)),'v78 energy arithmetic');
    | end
  function monitor_hp_partition_v79(u,p,old,y):
    | function monitor_hp_partition_v79(u,p,old,y)
    | %#codegen
    | % Necessary temperature-dependent HP integral bounds, not equipment calibration.
    | monitor_energy_commit_v78(u,p,old,y);
    | Te=subiv(subiv(P(p(12)),P(p(13))),P(p(14)));
    | A=muliv(P(p(15)),addiv(Te,P(273.15)));
    | floor=addiv(P(p(19)),P(p(20)));
    | for j=1:y(13)
    |     z=y(100+80*(j-1)+(1:80));
    |     heat=z(32:33)';source=z(34:35)';work=z(36:37)';
    |     if z(24)==0
    |         assert(all(source==0)&&all(work==0),'v79 OFF HP energies');
    |         continue;
    |     end
    |     % Held affine TES flow is monotone. Its endpoint hull extrema therefore
    |     % bound all intermediate temperatures; no production flow/root call.
    |     E=[min(z(11),z(13)) max(z(12),z(14))];
    |     hot=addiv(addiv(P(p(2)),diviv(E,P(p(1)))),P(p(17)));
    |     hot=[max(floor(1),hot(1)) max(floor(2),hot(2))];
    |     lift=subiv(addiv(hot,P(p(18))),Te);
    |     assert(A(1)>0&&lift(1)>0,'v79 positive HP axes');
    |     % Source fraction decreases with lift; work fraction increases. Integral
    |     % means belong to these ranges for every positive segment duration.
    |     sf=[diviv(P(A(1)),addiv(P(A(1)),P(lift(2))))*[1;0] ...
    |         diviv(P(A(2)),addiv(P(A(2)),P(lift(1))))*[0;1]];
    |     wf=[diviv(P(lift(1)),addiv(P(A(2)),P(lift(1))))*[1;0] ...
    |         diviv(P(lift(2)),addiv(P(A(1)),P(lift(2))))*[0;1]];
    |     sb=muliv(heat,sf);wb=muliv(heat,wf);
    |     assert(source(1)<=sb(2)&&sb(1)<=source(2),'v79 source temperature partition');
    |     assert(work(1)<=wb(2)&&wb(1)<=work(2),'v79 compressor temperature partition');
    | end
    | end
    | function z=P(x),z=[x x];end
    | function z=addiv(x,y)
    | z=out([x(1)+y(1) x(2)+y(2)]);
    | end
    | function z=subiv(x,y)
    | z=out([x(1)-y(2) x(2)-y(1)]);
    | end
    | function z=muliv(x,y)
    | if all(x==0)||all(y==0),z=[0 0];return;end
    | v=[x(1)*y(1) x(1)*y(2) x(2)*y(1) x(2)*y(2)];z=out([min(v) max(v)]);
    | end
    | function z=diviv(x,y)
    | assert(y(1)>0,'v79 positive denominator');
    | v=[x(1)/y(1) x(1)/y(2) x(2)/y(1) x(2)/y(2)];z=out([min(v) max(v)]);
    | end
    | function z=out(x)
    | z=[x(1)-2*eps(x(1)) x(2)+2*eps(x(2))];assert(all(isfinite(z)),'v79 HP bound arithmetic');
    | end
